simulink model "Lab2_2_1_1_4_BE_FF"  (R2024b)
settings: Solver=VariableStepAuto  StartTime=0.0  StopTime=3  FixedStep=1e-03  RelTol=1e-1
undefined symbols (not defined in the file): BEMF_comp, DiscIntNeverNeededParam, drv, dspblkCoreblockFVToolHelper, gbox, gcbh, Inertia_comp, Kd, Ki, Kp, mld, mot, N2Beq, rads2rpm, rpm2rads, sens, T2, Tau_sf, TL
libraries: SignalEditorBlockLib x1
settings Model: SimulationMode=external  ExtModeTrigDuration=45001  Creator=lenovo  LastModifiedBy=liliy
settings SolverCC: ZeroCrossAlgorithm=Adaptive
settings DataIOCC: ReturnWorkspaceOutputs=off
settings DebuggingCC: IgnoredZcDiagnostic=none
settings HardwareCC: ProdBitPerLong=64  ProdHWDeviceType=Intel->x86-64 (Linux 64)
settings RTWCC: Description=Simulink Desktop Real-Time  SystemTargetFile=sldrt.tlc  TemplateMakefile=sldrt.tmf  RTWCompilerOptimization=on
settings CodeAppCC: MaxIdLength=95
settings SimulinkDesktopRealTimeCC: TargetLibSuffix=_sldrt.a  TargetPreCompLibLocation=C:\Program Files\MATLAB\R2024b\toolbox\sldrt\lib\win64  ParMdlRefBuildCompliant=on

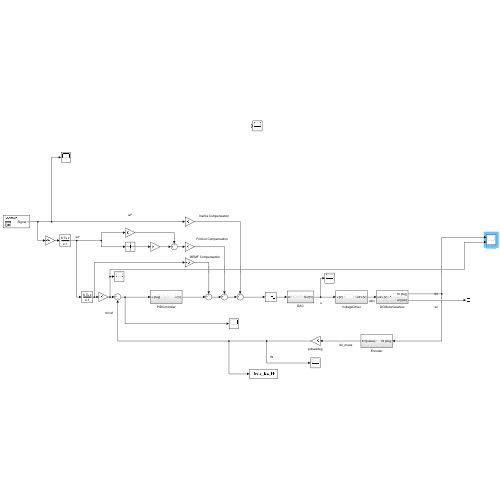
[thumbnail: Simulink's stored preview of the top-level diagram]
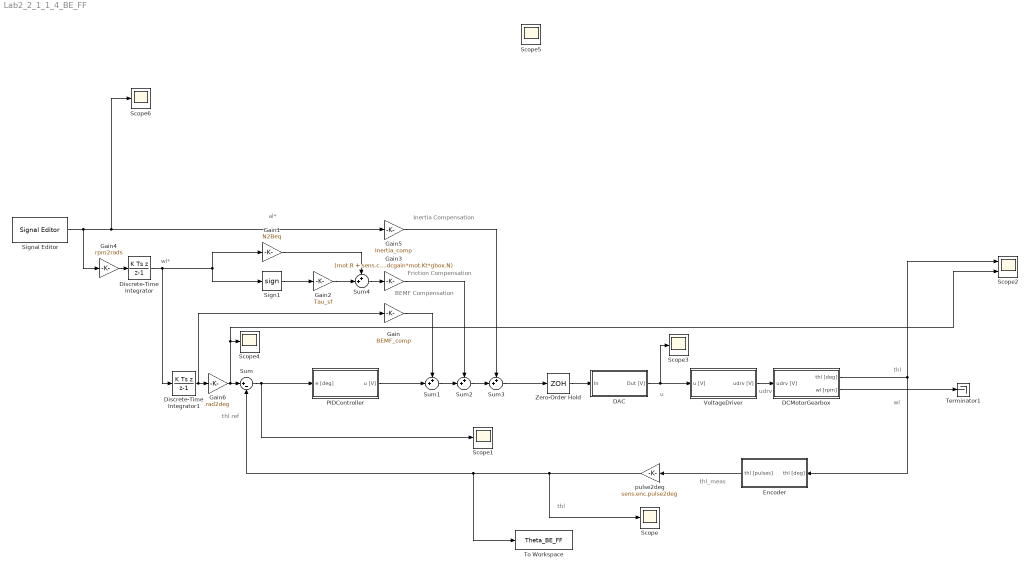
== system Lab2_2_1_1_4_BE_FF ==
  note: thl
  note: thl ref
  note: thl
  note: wl
  note: u
  note: thl_meas
  note: udrv
  note: BEMF Compensation
  note: Inertia Compensation
  note: al*
  note: Friction Compensation
  note: wl*
  DAC : Subsystem
  DCMotorGearbox : Subsystem
  Discrete-Time Integrator : DiscreteIntegrator  IntegratorMethod=Integration: Backward Euler  SampleTime=T2  ICPrevOutput=DiscIntNeverNeededParam  ICPrevScaledInput=DiscIntNeverNeededParam
  Discrete-Time Integrator1 : DiscreteIntegrator  IntegratorMethod=Integration: Backward Euler  SampleTime=T2  ICPrevOutput=DiscIntNeverNeededParam  ICPrevScaledInput=DiscIntNeverNeededParam
  Encoder : Subsystem
  Gain : Gain  Gain=BEMF_comp
  Gain1 : Gain  Gain=N2Beq
  Gain2 : Gain  Gain=Tau_sf
  Gain3 : Gain  Gain=(mot.R + sens.curr.Rs)/(drv.dcgain*mot.Kt*gbox.N)
  Gain4 : Gain  Gain=rpm2rads
  Gain5 : Gain  Gain=Inertia_comp
  Gain6 : Gain  Gain=rad2deg
  PIDController : Subsystem
  Scope{,1,3..6} (6 alike) : Scope
  Scope2 : Scope  NumInputPorts=2
  Sign1 : Signum
  Signal Editor : SignalEditorBlockLib/Signal Editor  FileName=Aprofile.mat  ActiveScenario=Scenario  ActiveSignal=Signal 1  IsBus=off  OutputBusObjectStr=Bus: BusObject  SampleTime=T2  Interpolate=off  ZeroCross=off  OutputAfterFinalValue=Setting to zero  Unit=inherit  PreserveSignalName=on  ApplySigPropsToAllScenarios=on  ApplySigPropsToAllSignals=off
  Sum : Sum  Inputs=|+-
  Sum{1..4} (4 alike) : Sum  Inputs=++|
  Terminator1 : Terminator
  To Workspace : ToWorkspace  VariableName=Theta_BE_FF  SaveFormat=Structure With Time  SampleTime=0.001
  VoltageDriver : Subsystem
  Zero-Order Hold : ZeroOrderHold  SampleTime=T2
  pulse2deg : Gain  Gain=sens.enc.pulse2deg
  wires:
  pulse2deg/1 -> Scope/1, To Workspace/1, Sum/2
  Sum/1 -> PIDController/1(e [deg]), Scope1/1
  Zero-Order Hold/1 -> DAC/1(In)
  DCMotorGearbox/2(wl [rpm]) -> Terminator1/1
  DCMotorGearbox/1(thl [deg]) -> Encoder/1(thl [deg]), Scope2/1
  VoltageDriver/1(udrv [V]) -> DCMotorGearbox/1(udrv [V])
  DAC/1(Out [V]) -> VoltageDriver/1(u [V]), Scope3/1
  Encoder/1(thl [pulses]) -> pulse2deg/1
  Gain5/1 -> Sum3/1
  Gain/1 -> Sum1/1
  Discrete-Time Integrator/1 -> Discrete-Time Integrator1/1, Gain1/1, Sign1/1
  Gain2/1 -> Sum4/2
  Sign1/1 -> Gain2/1
  Gain1/1 -> Sum4/1
  Sum4/1 -> Gain3/1
  Gain3/1 -> Sum2/1
  Signal Editor/1 -> Gain4/1, Scope6/1, Gain5/1
  PIDController/1(u [V]) -> Sum1/2
  Sum1/1 -> Sum2/2
  Sum2/1 -> Sum3/2
  Sum3/1 -> Zero-Order Hold/1
  Gain4/1 -> Discrete-Time Integrator/1
  Discrete-Time Integrator1/1 -> Gain/1, Gain6/1
  Gain6/1 -> Scope2/2, Scope4/1, Sum/1

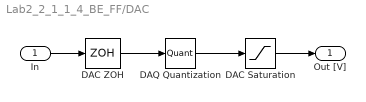
== system Lab2_2_1_1_4_BE_FF/DAC ==
  In : Inport
  DAC Saturation : Saturate  UpperLimit=10  LowerLimit=-10
  DAC ZOH : ZeroOrderHold  SampleTime=1e-03
  DAQ Quantization : Quantizer  QuantizationInterval=daq.dac.q
  Out [V] : Outport
  wires:
  DAC Saturation/1 -> Out [V]/1
  DAQ Quantization/1 -> DAC Saturation/1
  DAC ZOH/1 -> DAQ Quantization/1
  In/1 -> DAC ZOH/1

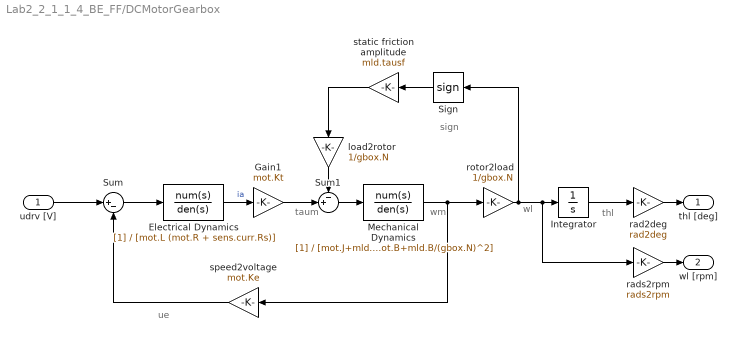
== system Lab2_2_1_1_4_BE_FF/DCMotorGearbox ==
  note: sign
  note: taum
  note: ue
  note: thl
  note: wm
  note: wl
  udrv [V] : Inport
  Electrical Dynamics : TransferFcn  Denominator=[mot.L (mot.R + sens.curr.Rs)]
  Gain1 : Gain  Gain=mot.Kt
  Integrator : Integrator
  Mechanical Dynamics : TransferFcn  Denominator=[mot.J+mld.J/(gbox.N)^2 mot.B+mld.B/(gbox.N)^2]
  Sign : Signum
  Sum : Sum  Inputs=|+-
  Sum1 : Sum  Inputs=-+|
  load2rotor : Gain  Gain=1/gbox.N
  rad2deg : Gain  Gain=rad2deg
  rads2rpm : Gain  Gain=rads2rpm
  rotor2load : Gain  Gain=1/gbox.N
  speed2voltage : Gain  Gain=mot.Ke
  static friction amplitude : Gain  Gain=mld.tausf
  thl [deg] : Outport
  wl [rpm] : Outport  Port=2
  wires:
  Gain1/1 -> Sum1/2
  Electrical Dynamics/1 -> Gain1/1  "ia"
  Sum1/1 -> Mechanical Dynamics/1
  speed2voltage/1 -> Sum/2
  load2rotor/1 -> Sum1/1
  Sum/1 -> Electrical Dynamics/1
  Sign/1 -> static friction amplitude/1
  static friction amplitude/1 -> load2rotor/1
  rotor2load/1 -> rads2rpm/1, Integrator/1, Sign/1
  rad2deg/1 -> thl [deg]/1
  udrv [V]/1 -> Sum/1
  Integrator/1 -> rad2deg/1
  Mechanical Dynamics/1 -> rotor2load/1, speed2voltage/1
  rads2rpm/1 -> wl [rpm]/1

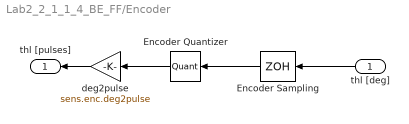
== system Lab2_2_1_1_4_BE_FF/Encoder ==
  thl [deg] : Inport
  Encoder Quantizer : Quantizer  QuantizationInterval=360/sens.enc.ppr
  Encoder Sampling : ZeroOrderHold  SampleTime=T2
  deg2pulse : Gain  Gain=sens.enc.deg2pulse
  thl [pulses] : Outport
  wires:
  thl [deg]/1 -> Encoder Sampling/1
  deg2pulse/1 -> thl [pulses]/1
  Encoder Sampling/1 -> Encoder Quantizer/1
  Encoder Quantizer/1 -> deg2pulse/1

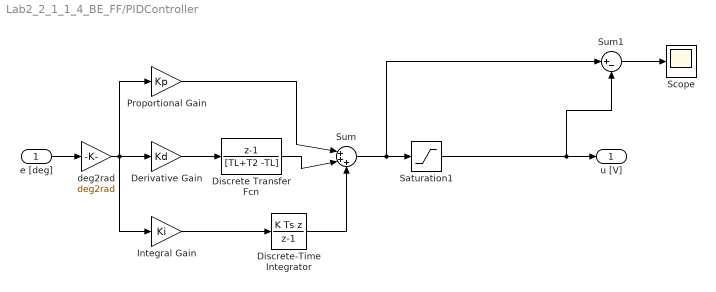
== system Lab2_2_1_1_4_BE_FF/PIDController ==
  e [deg] : Inport
  Derivative Gain : Gain  Gain=Kd
  Discrete Transfer Fcn : DiscreteTransferFcn  LoadFcn=dspblkCoreblockFVToolHelper(gcbh,'load');  Numerator=[1 -1]  Denominator=[TL+T2 -TL]
      settings: CopyFcn=dspblkCoreblockFVToolHelper(gcbh,'copy');  DeleteFcn=dspblkCoreblockFVToolHelper(gcbh,'close');  ModelCloseFcn=dspblkCoreblockFVToolHelper(gcbh,'close');  PreSaveFcn=dspblkCoreblockFVToolHelper(gcbh,'presave');  PostSaveFcn=dspblkCoreblockFVToolHelper(gcbh,'postsave');  CloseFcn=dspblkCoreblockFVToolHelper(gcbh,'close');
  Discrete-Time Integrator : DiscreteIntegrator  IntegratorMethod=Integration: Backward Euler  SampleTime=T2  ICPrevOutput=DiscIntNeverNeededParam  ICPrevScaledInput=DiscIntNeverNeededParam
  Integral Gain : Gain  Gain=Ki
  Proportional Gain : Gain  Gain=Kp
  Saturation1 : Saturate  UpperLimit=12  LowerLimit=-12
  Scope : Scope
  Sum : Sum  Inputs=|+++
  Sum1 : Sum  Inputs=|+-
  deg2rad : Gain  Gain=deg2rad
  u [V] : Outport
  wires:
  Saturation1/1 -> Sum1/2, u [V]/1
  Sum1/1 -> Scope/1
  deg2rad/1 -> Integral Gain/1, Derivative Gain/1, Proportional Gain/1
  e [deg]/1 -> deg2rad/1
  Proportional Gain/1 -> Sum/1
  Discrete Transfer Fcn/1 -> Sum/2
  Sum/1 -> Sum1/1, Saturation1/1
  Derivative Gain/1 -> Discrete Transfer Fcn/1
  Discrete-Time Integrator/1 -> Sum/3
  Integral Gain/1 -> Discrete-Time Integrator/1

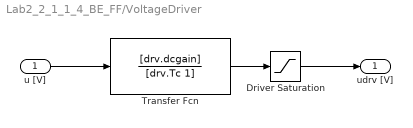
== system Lab2_2_1_1_4_BE_FF/VoltageDriver ==
  u [V] : Inport
  Driver Saturation : Saturate  UpperLimit=12  LowerLimit=-12
  Transfer Fcn : TransferFcn  Numerator=[drv.dcgain]  Denominator=[drv.Tc 1]
  udrv [V] : Outport
  wires:
  u [V]/1 -> Transfer Fcn/1
  Transfer Fcn/1 -> Driver Saturation/1
  Driver Saturation/1 -> udrv [V]/1
